simulink model "plant_model"  (R2024b)
settings: Solver=ode4  StartTime=0.0  StopTime=0.1  FixedStep=1e-6  RelTol=1e-3
libraries: spsSeriesRLCBranchLib x11, fuzblock x7, spsPWMGeneratorDCDCLib x7, spsFirstOrderFilterLib x4, spsIGBTDiodeLib x4, spsControlledVoltageSourceLib x3, spsCurrentMeasurementLib x3, spsGroundLib x3, spsVoltageMeasurementLib x3, spsIdealSwitchLib x2, SignalEditorBlockLib x2, spsDiodeLib x1
settings Model: Creator=Crisplan  LastModifiedBy=Crisplan
settings DataIOCC: ExternalInput=Input_Signals  LoadExternalInput=on

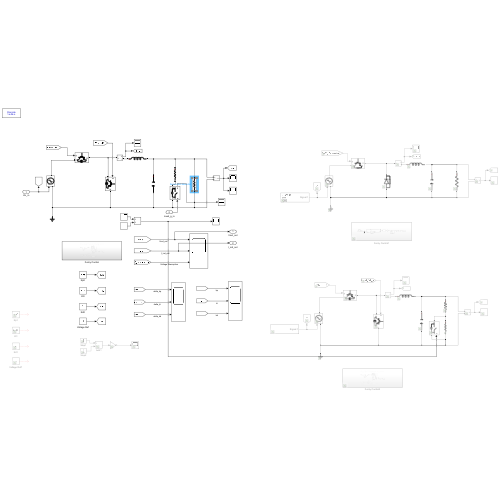
[thumbnail: Simulink's stored preview of the top-level diagram]
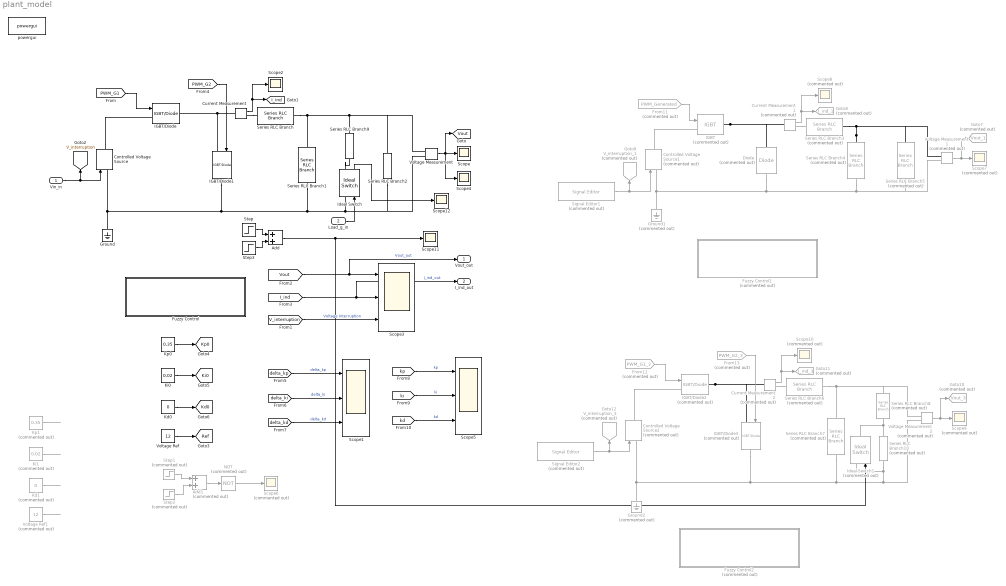
== system plant_model ==
  Vin_in : Inport
  Load_g_in : Inport  Port=2
  Add : Sum
  Add1 : Sum  Commented=on
  Controlled Voltage Source : spsControlledVoltageSourceLib/Controlled Voltage Source  Initialize=on  Source_Type=DC  Amplitude=0  Phase=0  Frequency=0  Measurements=None
  Controlled Voltage Source1 : spsControlledVoltageSourceLib/Controlled Voltage Source  Commented=on  Initialize=on  Source_Type=DC  Amplitude=0  Phase=0  Frequency=0  Measurements=None
  Controlled Voltage Source2 : spsControlledVoltageSourceLib/Controlled Voltage Source  Commented=on  Initialize=on  Source_Type=DC  Amplitude=0  Phase=0  Frequency=0  Measurements=None
  Current Measurement : spsCurrentMeasurementLib/Current Measurement  PhasorSimulation=off  OutputType=Complex  PSBequivalent=0
  Current Measurement1 : spsCurrentMeasurementLib/Current Measurement  Commented=on  PhasorSimulation=off  OutputType=Complex  PSBequivalent=0
  Current Measurement2 : spsCurrentMeasurementLib/Current Measurement  Commented=on  PhasorSimulation=off  OutputType=Complex  PSBequivalent=0
  Diode : spsDiodeLib/Diode  Commented=on  Ron=0.001  Lon=0  Vf=0.8  IC=0  UseSnubber=0  Rs=500  Cs=250e-9  Measurements=off
  From11 : From  Commented=on  GotoTag=PWM_Generated  TagVisibility=global
  From12 : From  Commented=on  GotoTag=PWM_G1_3  TagVisibility=global
  From13 : From  Commented=on  GotoTag=PWM_G2_3  TagVisibility=global
  Fuzzy Control : Subsystem
  Fuzzy Control1 : Subsystem  Commented=on
  Fuzzy Control2 : Subsystem  Commented=on
  Goto10 : Goto  Commented=on  GotoTag=Vout_3  TagVisibility=global
  Goto11 : Goto  Commented=on  GotoTag=I_ind_3  TagVisibility=global
  Goto12 : Goto  Commented=on  GotoTag=V_interruption_3  TagVisibility=global
  Goto7 : Goto  Commented=on  GotoTag=Vout_1  TagVisibility=global
  Goto8 : Goto  Commented=on  GotoTag=I_ind_1  TagVisibility=global
  Goto9 : Goto  Commented=on  GotoTag=V_interruption_1  TagVisibility=global
  Ground : spsGroundLib/Ground  LConnTagsString=a
  Ground1 : spsGroundLib/Ground  Commented=on  LConnTagsString=a
  Ground2 : spsGroundLib/Ground  Commented=on  LConnTagsString=a
  IGBT : spsIGBTLib/IGBT  Commented=on  Ron=0.001  Lon=0  Vf=1  Tf=1e-6  Tt=2e-6  IC=0  Rs=1e5  Cs=inf  Measurements=off
  IGBT/Diode : spsIGBTDiodeLib/IGBT//Diode  Ron=1e-3  Rs=1e5  Cs=inf  Measurements=off
  IGBT/Diode1 : spsIGBTDiodeLib/IGBT//Diode  Ron=1e-3  Rs=1e5  Cs=inf  Measurements=off
  IGBT/Diode2 : spsIGBTDiodeLib/IGBT//Diode  Commented=on  Ron=1e-3  Rs=1e5  Cs=inf  Measurements=off
  IGBT/Diode3 : spsIGBTDiodeLib/IGBT//Diode  Commented=on  Ron=1e-3  Rs=1e5  Cs=inf  Measurements=off
  Ideal Switch : spsIdealSwitchLib/Ideal Switch  Ron=1e-6  Lon=0  IC=0  Rs=1e5  Cs=inf  Measurements=on
  Ideal Switch1 : spsIdealSwitchLib/Ideal Switch  Commented=on  Ron=0.001  Lon=0  IC=0  Rs=1e5  Cs=inf  Measurements=off
  Kd0 : Constant  Value=0  SampleTime=1e-4
  Kd1 : Constant  Commented=on  Value=0  SampleTime=1e-4
  Ki0 : Constant  Value=0.02  SampleTime=1e-4
  Ki1 : Constant  Commented=on  Value=0.02  SampleTime=1e-4
  Kp0 : Constant  Value=0.35  SampleTime=1e-4
  Kp1 : Constant  Commented=on  Value=0.35  SampleTime=1e-4
  NOT : Logic  Commented=on  Operator=NOT  IconShape=distinctive  AllPortsSameDT=off  OutDataTypeStr=boolean
  Scope{,2,4,11..12} (5 alike) : Scope
  Scope1 : Scope  NumInputPorts=3
  Scope{6..10} (5 alike) : Scope  Commented=on
  Scope3 : Scope  NumInputPorts=3
  Scope5 : Scope  NumInputPorts=3
  Series RLC Branch : spsSeriesRLCBranchLib/Series RLC Branch  LConnTagsString=__new0  RConnTagsString=__new0  BranchType=L  Resistance=1  Inductance=0.015  SetiL0=off  InitialCurrent=0  Capacitance=1e-6  Setx0=off  InitialVoltage=0  Measurements=None
  Series RLC Branch1 : spsSeriesRLCBranchLib/Series RLC Branch  LConnTagsString=__new0  RConnTagsString=__new0  BranchType=C  Resistance=1  Inductance=1e-3  SetiL0=off  InitialCurrent=0  Capacitance=50e-6  Setx0=off  InitialVoltage=0  Measurements=None
  Series RLC Branch10 : spsSeriesRLCBranchLib/Series RLC Branch  Commented=on  LConnTagsString=__new0  RConnTagsString=__new0  BranchType=R  Resistance=2  Inductance=1e-3  SetiL0=off  InitialCurrent=0  Capacitance=1e-6  Setx0=off  InitialVoltage=0  Measurements=None
  Series RLC Branch2 : spsSeriesRLCBranchLib/Series RLC Branch  LConnTagsString=__new0  RConnTagsString=__new0  BranchType=R  Resistance=10  Inductance=1e-3  SetiL0=off  InitialCurrent=0  Capacitance=1e-6  Setx0=off  InitialVoltage=0  Measurements=None
  Series RLC Branch3 : spsSeriesRLCBranchLib/Series RLC Branch  Commented=on  LConnTagsString=__new0  RConnTagsString=__new0  BranchType=L  Resistance=1  Inductance=0.015  SetiL0=off  InitialCurrent=0  Capacitance=1e-6  Setx0=off  InitialVoltage=0  Measurements=None
  Series RLC Branch4 : spsSeriesRLCBranchLib/Series RLC Branch  Commented=on  LConnTagsString=__new0  RConnTagsString=__new0  BranchType=C  Resistance=1  Inductance=1e-3  SetiL0=off  InitialCurrent=0  Capacitance=50e-6  Setx0=off  InitialVoltage=0  Measurements=None
  Series RLC Branch5 : spsSeriesRLCBranchLib/Series RLC Branch  Commented=on  LConnTagsString=__new0  RConnTagsString=__new0  BranchType=R  Resistance=10  Inductance=1e-3  SetiL0=off  InitialCurrent=0  Capacitance=1e-6  Setx0=off  InitialVoltage=0  Measurements=None
  Series RLC Branch6 : spsSeriesRLCBranchLib/Series RLC Branch  Commented=on  LConnTagsString=__new0  RConnTagsString=__new0  BranchType=L  Resistance=1  Inductance=0.015  SetiL0=off  InitialCurrent=0  Capacitance=1e-6  Setx0=off  InitialVoltage=0  Measurements=None
  Series RLC Branch7 : spsSeriesRLCBranchLib/Series RLC Branch  Commented=on  LConnTagsString=__new0  RConnTagsString=__new0  BranchType=C  Resistance=1  Inductance=1e-3  SetiL0=off  InitialCurrent=0  Capacitance=50e-6  Setx0=off  InitialVoltage=0  Measurements=None
  Series RLC Branch8 : spsSeriesRLCBranchLib/Series RLC Branch  Commented=on  LConnTagsString=__new0  RConnTagsString=__new0  BranchType=R  Resistance=10  Inductance=1e-3  SetiL0=off  InitialCurrent=0  Capacitance=1e-6  Setx0=off  InitialVoltage=0  Measurements=None
  Series RLC Branch9 : spsSeriesRLCBranchLib/Series RLC Branch  LConnTagsString=__new0  RConnTagsString=__new0  BranchType=R  Resistance=10  Inductance=1e-3  SetiL0=off  InitialCurrent=0  Capacitance=1e-6  Setx0=off  InitialVoltage=0  Measurements=None
  Signal Editor1 : SignalEditorBlockLib/Signal Editor  Commented=on  FileName=Vin_signal.mat  ActiveScenario=Scenario  ActiveSignal=Voltage Interruption  IsBus=off  OutputBusObjectStr=Bus: BusObject  SampleTime=0  Interpolate=off  ZeroCross=off  OutputAfterFinalValue=Setting to zero  Unit=inherit  PreserveSignalName=on  ApplySigPropsToAllScenarios=on  ApplySigPropsToAllSignals=off
  Signal Editor2 : SignalEditorBlockLib/Signal Editor  Commented=on  FileName=data\Vin.mat  ActiveScenario=Scenario  ActiveSignal=Voltage Interruption  IsBus=off  OutputBusObjectStr=Bus: BusObject  SampleTime=0  Interpolate=off  ZeroCross=off  OutputAfterFinalValue=Setting to zero  Unit=inherit  PreserveSignalName=on  ApplySigPropsToAllScenarios=on  ApplySigPropsToAllSignals=off
  Step : Step  Time=0  SampleTime=0
  Step1 : Step  Commented=on  Time=0.02  SampleTime=0
  Step2 : Step  Commented=on  Time=0.07  After=-1  SampleTime=0
  Step3 : Step  Time=0.02  After=-1  SampleTime=0
  Voltage Measurement : spsVoltageMeasurementLib/Voltage Measurement  PhasorSimulation=off  OutputType=Complex  PSBequivalent=0
  Voltage Measurement1 : spsVoltageMeasurementLib/Voltage Measurement  Commented=on  PhasorSimulation=off  OutputType=Complex  PSBequivalent=0
  Voltage Measurement2 : spsVoltageMeasurementLib/Voltage Measurement  Commented=on  PhasorSimulation=off  OutputType=Complex  PSBequivalent=0
  Voltage Ref : Constant  Value=12  SampleTime=1e-4
  Voltage Ref1 : Constant  Commented=on  Value=12  SampleTime=1e-4
  powergui : spspowerguiLib/powergui  Priority=1  SimulationMode=Discrete  SampleTime=1e-6  frequency=60  Iterations=50  frequencyindice=0  Pbase=100e6  ErrMax=1e-4  UnitsV=kV  UnitsW=MW  buscounter=0  FunctionMessages=off  echomessages=off  EnableUseOfTLC=off  CurrentSourceSwitches=off  DisableSnubberDevices=off  DisableRonSwitches=off  DisableVfSwitches=off  DisplayEquations=off  AutomaticDiscreteSolvers=off  SolverType=Tustin/Backward Euler (TBE)  Interpol=off  ExternalGateDelay=off  methode=off  Ts=100  x0status=blocks  SPID=on  SwTol=0  HookPort=off  NonlinearTolerance=1e-4  nMaxIteration=100  ContinueOnMaxIteration=off  RestoreLinks=warning  ResistiveCurrentMeasurement=off  Frange=[0:2:500]  Ylog=off  Xlog=on  ShowGrid=off  save=off  variable=ZData  structure=0  ZoomFFT=off  StartTime=0.0  cycles=1  DisplayStyle=1  fundamental=60  FreqAxis=off  MaxFrequency=1000  frequencyindicesteady=1  RmsSteady=1  display=off
  Vout_out : Outport
  I_ind_out : Outport  Port=2
  tag scope: I_ind=global, Kd0=global, Ki0=global, Kp0=global, Ref=global, V_interruption=global, Vout=global
  wires:
  [I_ind] -> Scope3/2, I_ind_out/1  "I_ind_out"
  Voltage Measurement/1 -> Scope4/1, [Vout], Scope/1
  [V_interruption] -> Scope3/3  "Voltage Interruption"
  Vin_in/1 -> [V_interruption], Controlled Voltage Source/1
  [Vout] -> Scope3/1, Vout_out/1  "Vout_out"
  [PWM_G1] -> IGBT/Diode/1
  Current Measurement/1 -> Scope2/1, [I_ind]
  Voltage Ref/1 -> [Ref]
  Kp0/1 -> [Kp0]
  Ki0/1 -> [Ki0]
  Kd0/1 -> [Kd0]
  [PWM_G2] -> IGBT/Diode1/1
  [delta_ki] -> Scope1/2  "delta_ki"
  [delta_kp] -> Scope1/1  "delta_kp"
  [delta_kd] -> Scope1/3  "delta_kd"
  [kp] -> Scope5/1  "kp"
  [ki] -> Scope5/2  "ki"
  [kd] -> Scope5/3  "kd"
  Step1/1 -> Add1/1
  Step2/1 -> Add1/2
  Add1/1 -> NOT/1
  NOT/1 -> Scope6/1
  Signal Editor1/1 -> Goto9/1, Controlled Voltage Source1/1
  Voltage Measurement1/1 -> Goto7/1, Scope7/1
  From11/1 -> IGBT/1
  Current Measurement1/1 -> Scope8/1, Goto8/1
  Current Measurement2/1 -> Scope10/1, Goto11/1
  From13/1 -> IGBT/Diode3/1
  Voltage Measurement2/1 -> Goto10/1, Scope9/1
  From12/1 -> IGBT/Diode2/1
  Signal Editor2/1 -> Goto12/1, Controlled Voltage Source2/1
  Step/1 -> Add/1
  Step3/1 -> Add/2
  Kd1/1 -> ?
  Voltage Ref1/1 -> ?
  Kp1/1 -> ?
  Ki1/1 -> ?
  Add/1 -> Scope11/1, Ideal Switch1/1
  Ideal Switch/1 -> Scope12/1
  Load_g_in/1 -> Ideal Switch/1
  connections:
  Series RLC Branch9/LConn1 -- Series RLC Branch2/LConn1 -- Voltage Measurement/LConn1 -- Series RLC Branch1/LConn1 -- Series RLC Branch/RConn1
  Ground/LConn1 -- Series RLC Branch2/RConn1 -- Voltage Measurement/LConn2 -- Ideal Switch/LConn1 -- Series RLC Branch1/RConn1 -- IGBT/Diode1/RConn1 -- Controlled Voltage Source/LConn1
  Current Measurement/LConn1 -- IGBT/Diode1/LConn1 -- IGBT/Diode/RConn1
  IGBT/Diode/LConn1 -- Controlled Voltage Source/RConn1
  Current Measurement/RConn1 -- Series RLC Branch/LConn1
  Ground1/LConn1 -- Diode/LConn1 -- Voltage Measurement1/LConn2 -- Series RLC Branch5/RConn1 -- Series RLC Branch4/RConn1 -- Controlled Voltage Source1/LConn1
  Series RLC Branch4/LConn1 -- Series RLC Branch3/RConn1 -- Voltage Measurement1/LConn1 -- Series RLC Branch5/LConn1
  IGBT/RConn1 -- Diode/RConn1 -- Current Measurement1/LConn1
  IGBT/LConn1 -- Controlled Voltage Source1/RConn1
  Current Measurement1/RConn1 -- Series RLC Branch3/LConn1
  Series RLC Branch6/RConn1 -- Series RLC Branch7/LConn1 -- Voltage Measurement2/LConn1 -- Series RLC Branch8/LConn1
  Series RLC Branch10/RConn1 -- Ground2/LConn1 -- Controlled Voltage Source2/LConn1 -- IGBT/Diode3/RConn1 -- Series RLC Branch7/RConn1 -- Voltage Measurement2/LConn2 -- Ideal Switch1/LConn1
  IGBT/Diode2/RConn1 -- Current Measurement2/LConn1 -- IGBT/Diode3/LConn1
  IGBT/Diode2/LConn1 -- Controlled Voltage Source2/RConn1
  Current Measurement2/RConn1 -- Series RLC Branch6/LConn1
  Series RLC Branch10/LConn1 -- Series RLC Branch8/RConn1 -- Ideal Switch1/RConn1
  Ideal Switch/RConn1 -- Series RLC Branch9/RConn1

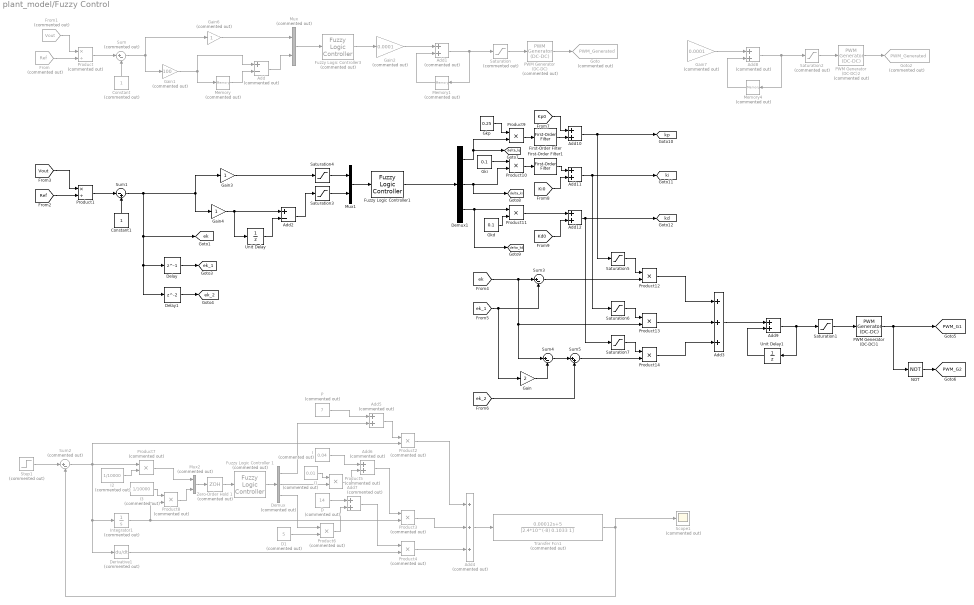
== system plant_model/Fuzzy Control ==
  Add : Sum  Commented=on  Inputs=+-
  Add{1,5..8} (5 alike) : Sum  Commented=on
  Add{9..12} (4 alike) : Sum
  Add2 : Sum  Inputs=+-
  Add3 : Sum  Inputs=+++
  Add4 : Sum  Commented=on  Inputs=+++
  Constant : Constant  Commented=on
  Constant1 : Constant  SampleTime=1e-4
  D : Constant  Commented=on  Value=14
  D1 : Constant  Commented=on  Value=5
  Delay : Delay  DelayLength=1  SampleTime=1e-4
  Delay1 : Delay  SampleTime=1e-4
  Demux : Demux  Commented=on  Outputs=3
  Demux1 : Demux  Outputs=3
  Derivative1 : Derivative  Commented=on
  First-Order Filter : spsFirstOrderFilterLib/First-Order Filter  FilterType=Lowpass  Tc=0.003  Ts=0  Initialize=on  Vac_Init=[0, 0, 60]  Vdc_Init=0  PlotResponse=off  FreqRange="[0,  200,  1]"
  First-Order Filter1 : spsFirstOrderFilterLib/First-Order Filter  FilterType=Lowpass  Tc=0.003  Ts=0  Initialize=on  Vac_Init=[0, 0, 60]  Vdc_Init=0  PlotResponse=off  FreqRange="[0,  200,  1]"
  From : From  Commented=on  GotoTag=Ref  TagVisibility=global
  From1 : From  Commented=on  GotoTag=Vout  TagVisibility=global
  Fuzzy Logic Controller 1 : fuzblock/Fuzzy Logic  Controller  Commented=on  FIS='FuzzyPID_Triangle_V1.fis'  OutputSampleNumber=101  DataType=double  FuzzifiedInputs=off  RuleFiringStrengths=off  RuleOutputs=off  AggregatedOutputs=off  SimulateUsing=Interpreted execution  OutOfRangeInputValueMessage=warning  NoRuleFiredMessage=warning  EmptyOutputFuzzySetMessage=warning
  Fuzzy Logic Controller1 : fuzblock/Fuzzy Logic  Controller  FIS=fuzzy_rules  OutputSampleNumber=101  DataType=double  FuzzifiedInputs=off  RuleFiringStrengths=off  RuleOutputs=off  AggregatedOutputs=off  SimulateUsing=Interpreted execution  OutOfRangeInputValueMessage=warning  NoRuleFiredMessage=warning  EmptyOutputFuzzySetMessage=warning
  Fuzzy Logic Controller3 : fuzblock/Fuzzy Logic  Controller  Commented=on  FIS=Fuzzy_1  OutputSampleNumber=101  DataType=double  FuzzifiedInputs=off  RuleFiringStrengths=off  RuleOutputs=off  AggregatedOutputs=off  SimulateUsing=Interpreted execution  OutOfRangeInputValueMessage=warning  NoRuleFiredMessage=warning  EmptyOutputFuzzySetMessage=warning
  Gain : Gain  Gain=2
  Gain1 : Gain  Commented=on  Gain=100
  Gain2 : Gain  Commented=on  Gain=0.0001
  Gain3 : Gain
  Gain4 : Gain
  Gain6 : Gain  Commented=on
  Gain7 : Gain  Commented=on  Gain=0.0001
  Gkd : Constant  Value=0.1  SampleTime=1e-4
  Gki : Constant  Value=0.1  SampleTime=1e-4
  Gkp : Constant  Value=0.25  SampleTime=1e-4
  Goto : Goto  Commented=on  GotoTag=PWM_Generated  TagVisibility=global
  Goto2 : Goto  Commented=on  GotoTag=PWM_Generated  TagVisibility=global
  I : Constant  Commented=on  Value=0.04
  I1 : Constant  Commented=on  Value=0.01
  I2 : Constant  Commented=on  Value=1/10000
  I3 : Constant  Commented=on  Value=1/10000
  Integrator1 : Integrator  Commented=on
  Memory : Memory  Commented=on  InheritSampleTime=on
  Memory1 : Memory  Commented=on  InheritSampleTime=on
  Memory4 : Memory  Commented=on  InheritSampleTime=on
  Mux : Mux  Commented=on  Inputs=2
  Mux1 : Mux  Inputs=2
  Mux2 : Mux  Commented=on  Inputs=2
  NOT : Logic  Operator=NOT  IconShape=distinctive  AllPortsSameDT=off  OutDataTypeStr=boolean
  P : Constant  Commented=on  Value=7
  PWM Generator (DC-DC) : spsPWMGeneratorDCDCLib/PWM Generator (DC-DC)  Commented=on  Fsw=5000  Ts=0
  PWM Generator (DC-DC)1 : spsPWMGeneratorDCDCLib/PWM Generator (DC-DC)  Fsw=1e4  Ts=0
  PWM Generator (DC-DC)2 : spsPWMGeneratorDCDCLib/PWM Generator (DC-DC)  Commented=on  Fsw=5000  Ts=0
  Product : Product  Commented=on  Inputs=*/
  Product1 : Product  Inputs=*/
  Product{9..14} (6 alike) : Product
  Product{2..8} (7 alike) : Product  Commented=on
  Saturation : Saturate  Commented=on  UpperLimit=1  LowerLimit=0
  Saturation1 : Saturate  UpperLimit=0.8  LowerLimit=0
  Saturation2 : Saturate  Commented=on  UpperLimit=1  LowerLimit=0
  Saturation3 : Saturate  UpperLimit=3  LowerLimit=-3
  Saturation4 : Saturate  UpperLimit=3  LowerLimit=-3
  Saturation5 : Saturate  UpperLimit=5  LowerLimit=-1
  Saturation6 : Saturate  UpperLimit=5  LowerLimit=-1
  Saturation7 : Saturate  UpperLimit=5  LowerLimit=-1
  Scope1 : Scope  Commented=on
  Step1 : Step  Commented=on  SampleTime=0
  Sum : Sum  Commented=on  Inputs=|+-
  Sum1 : Sum  Inputs=|-+
  Sum2 : Sum  Commented=on  Inputs=|+-
  Sum3 : Sum  Inputs=|+-
  Sum4 : Sum  Inputs=|+-
  Sum5 : Sum  Inputs=|++
  Transfer Fcn1 : TransferFcn  Commented=on  Numerator=[0.00012 5]  Denominator=[2.4*10^(-8) 0.1033 1]
  Unit Delay : UnitDelay  SampleTime=1e-4  HasFrameUpgradeWarning=on
  Unit Delay1 : UnitDelay  SampleTime=1e-4  HasFrameUpgradeWarning=on
  Zero-Order Hold 1 : ZeroOrderHold  Commented=on  SampleTime=-1
  tag scope: PWM_G1=global, PWM_G2=global, delta_kd=global, delta_ki=global, delta_kp=global, ek=global, ek_1=global, ek_2=global, kd=global, ki=global, kp=global
  wires:
  From1/1 -> Product/1
  Product/1 -> Sum/1
  Add/1 -> Mux/2
  Saturation/1 -> PWM Generator (DC-DC)/1
  Add1/1 -> Saturation/1, Memory1/1
  Fuzzy Logic Controller3/1 -> Gain2/1
  Gain1/1 -> Memory/1, Add/1
  Sum/1 -> Gain6/1, Gain1/1
  Gain2/1 -> Add1/1
  Memory1/1 -> Add1/2
  PWM Generator (DC-DC)/1 -> Goto/1
  Memory/1 -> Add/2
  Constant/1 -> Sum/2
  From/1 -> Product/2
  Mux/1 -> Fuzzy Logic Controller3/1
  Gain6/1 -> Mux/1
  Product1/1 -> Sum1/1
  Constant1/1 -> Sum1/2
  [Vout] -> Product1/1
  [Ref] -> Product1/2
  I2/1 -> Product7/2
  Zero-Order Hold 1/1 -> Fuzzy Logic Controller 1/1
  Add7/1 -> Product4/1
  Product7/1 -> Mux2/1
  Product4/1 -> Add4/3
  Product6/1 -> Add7/2
  Product3/1 -> Add4/2
  Transfer Fcn1/1 -> Scope1/1, Sum2/2
  Add6/1 -> Product3/1
  Fuzzy Logic Controller 1/1 -> Demux/1
  Step1/1 -> Sum2/1
  I3/1 -> Product8/1
  I1/1 -> Product5/1
  Demux/1 -> Add5/2
  I/1 -> Add6/1
  Product8/1 -> Mux2/2
  Add4/1 -> Transfer Fcn1/1
  Integrator1/1 -> Product8/2, Product3/2
  Demux/3 -> Product6/1
  Sum2/1 -> Derivative1/1, Integrator1/1, Product7/1, Product2/2
  Mux2/1 -> Zero-Order Hold 1/1
  Product2/1 -> Add4/1
  Demux/2 -> Product5/2
  P/1 -> Add5/1
  D/1 -> Add7/1
  Add5/1 -> Product2/1
  Product5/1 -> Add6/2
  D1/1 -> Product6/2
  Derivative1/1 -> Product4/2
  Saturation2/1 -> PWM Generator (DC-DC)2/1
  ? -> Gain7/1
  Memory4/1 -> Add8/2
  Add8/1 -> Saturation2/1, Memory4/1
  Gain7/1 -> Add8/1
  PWM Generator (DC-DC)2/1 -> Goto2/1
  Fuzzy Logic Controller1/1 -> Demux1/1
  Delay/1 -> [ek_1]
  Delay1/1 -> [ek_2]
  Gkp/1 -> Product9/1
  Demux1/1 -> [delta_kp], Product9/2
  Gki/1 -> Product10/1
  Demux1/2 -> [delta_ki], Product10/2
  Gkd/1 -> Product11/2
  Demux1/3 -> [delta_kd], Product11/1
  [ek] -> Sum4/1, Product13/2, Sum3/1
  [ek_1] -> Gain/1, Sum3/2
  Sum3/1 -> Product12/2
  Gain/1 -> Sum4/2
  Sum4/1 -> Sum5/1
  [ek_2] -> Sum5/2
  Sum5/1 -> Product14/2
  Product12/1 -> Add3/1
  Product13/1 -> Add3/2
  Product14/1 -> Add3/3
  Add3/1 -> Add9/1
  Add9/1 -> Unit Delay1/1, Saturation1/1
  [Kp0] -> Add10/1
  [Ki0] -> Add11/2
  Product11/1 -> Add12/1
  [Kd0] -> Add12/2
  Add10/1 -> [kp], Saturation5/1
  Add11/1 -> [ki], Saturation6/1
  Add12/1 -> [kd], Saturation7/1
  Saturation1/1 -> PWM Generator (DC-DC)1/1
  PWM Generator (DC-DC)1/1 -> NOT/1, [PWM_G1]
  NOT/1 -> [PWM_G2]
  Sum1/1 -> Gain4/1, Gain3/1, Delay1/1, Delay/1, [ek]
  Mux1/1 -> Fuzzy Logic Controller1/1
  Gain4/1 -> Unit Delay/1, Add2/1
  Add2/1 -> Saturation3/1
  Unit Delay1/1 -> Add9/2
  Product9/1 -> First-Order Filter/1
  First-Order Filter/1 -> Add10/2
  Product10/1 -> First-Order Filter1/1
  First-Order Filter1/1 -> Add11/1
  Saturation3/1 -> Mux1/2
  Gain3/1 -> Saturation4/1
  Saturation4/1 -> Mux1/1
  Saturation5/1 -> Product12/1
  Saturation6/1 -> Product13/1
  Saturation7/1 -> Product14/1
  Unit Delay/1 -> Add2/2

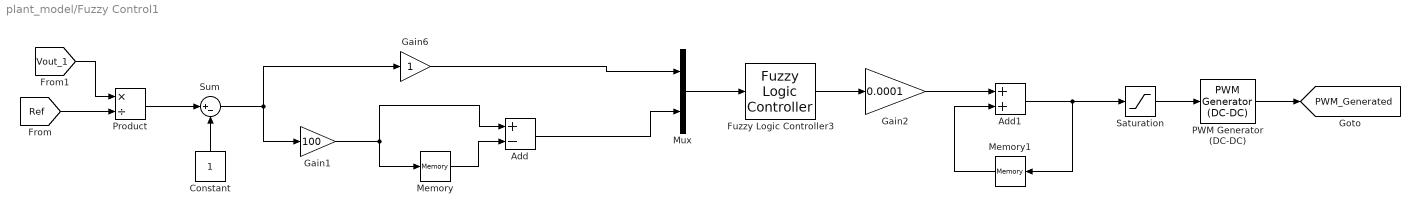
== system plant_model/Fuzzy Control1 ==
  Add : Sum  Inputs=+-
  Add1 : Sum
  Constant : Constant
  Fuzzy Logic Controller3 : fuzblock/Fuzzy Logic  Controller  FIS=Fuzzy_1  OutputSampleNumber=101  DataType=double  FuzzifiedInputs=off  RuleFiringStrengths=off  RuleOutputs=off  AggregatedOutputs=off  SimulateUsing=Interpreted execution  OutOfRangeInputValueMessage=warning  NoRuleFiredMessage=warning  EmptyOutputFuzzySetMessage=warning
  Gain1 : Gain  Gain=100
  Gain2 : Gain  Gain=0.0001
  Gain6 : Gain
  Memory : Memory  InheritSampleTime=on
  Memory1 : Memory  InheritSampleTime=on
  Mux : Mux  Inputs=2
  PWM Generator (DC-DC) : spsPWMGeneratorDCDCLib/PWM Generator (DC-DC)  Fsw=5000  Ts=0
  Product : Product  Inputs=*/
  Saturation : Saturate  UpperLimit=1  LowerLimit=0
  Sum : Sum  Inputs=|+-
  tag scope: PWM_Generated=global
  wires:
  [Vout_1] -> Product/1
  Product/1 -> Sum/1
  Saturation/1 -> PWM Generator (DC-DC)/1
  Add1/1 -> Saturation/1, Memory1/1
  Fuzzy Logic Controller3/1 -> Gain2/1
  Gain1/1 -> Memory/1, Add/1
  Sum/1 -> Gain6/1, Gain1/1
  Gain2/1 -> Add1/1
  Memory1/1 -> Add1/2
  PWM Generator (DC-DC)/1 -> [PWM_Generated]
  Memory/1 -> Add/2
  Constant/1 -> Sum/2
  [Ref] -> Product/2
  Mux/1 -> Fuzzy Logic Controller3/1
  Gain6/1 -> Mux/1
  Add/1 -> Mux/2

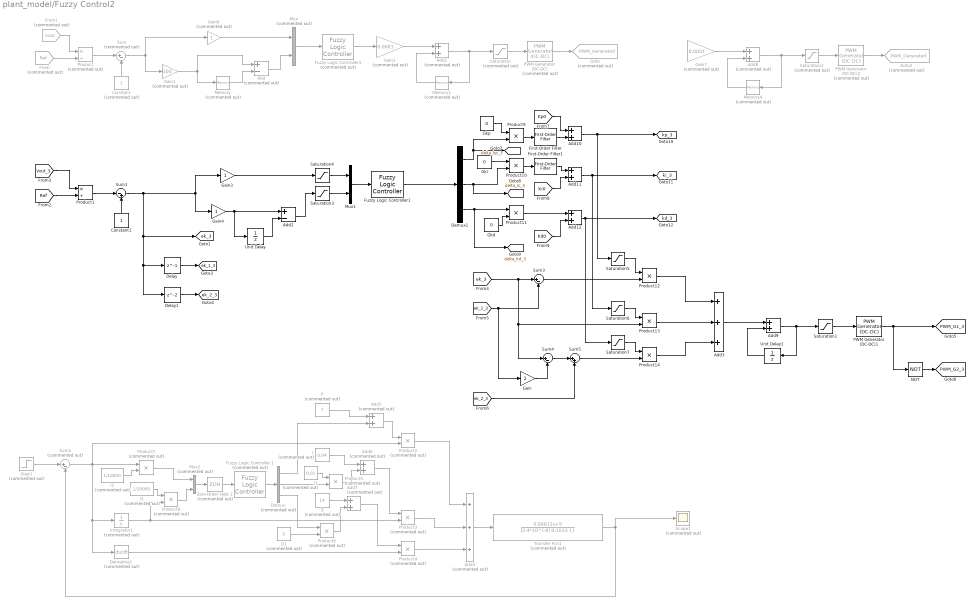
== system plant_model/Fuzzy Control2 ==
  Add : Sum  Commented=on  Inputs=+-
  Add{1,5..8} (5 alike) : Sum  Commented=on
  Add{9..12} (4 alike) : Sum
  Add2 : Sum  Inputs=+-
  Add3 : Sum  Inputs=+++
  Add4 : Sum  Commented=on  Inputs=+++
  Constant : Constant  Commented=on
  Constant1 : Constant  SampleTime=1e-4
  D : Constant  Commented=on  Value=14
  D1 : Constant  Commented=on  Value=5
  Delay : Delay  DelayLength=1  SampleTime=1e-4
  Delay1 : Delay  SampleTime=1e-4
  Demux : Demux  Commented=on  Outputs=3
  Demux1 : Demux  Outputs=3
  Derivative1 : Derivative  Commented=on
  First-Order Filter : spsFirstOrderFilterLib/First-Order Filter  FilterType=Lowpass  Tc=0.003  Ts=0  Initialize=on  Vac_Init=[0, 0, 60]  Vdc_Init=0  PlotResponse=off  FreqRange="[0,  200,  1]"
  First-Order Filter1 : spsFirstOrderFilterLib/First-Order Filter  FilterType=Lowpass  Tc=0.003  Ts=0  Initialize=on  Vac_Init=[0, 0, 60]  Vdc_Init=0  PlotResponse=off  FreqRange="[0,  200,  1]"
  From : From  Commented=on  GotoTag=Ref  TagVisibility=global
  From1 : From  Commented=on  GotoTag=Vout  TagVisibility=global
  Fuzzy Logic Controller 1 : fuzblock/Fuzzy Logic  Controller  Commented=on  FIS='FuzzyPID_Triangle_V1.fis'  OutputSampleNumber=101  DataType=double  FuzzifiedInputs=off  RuleFiringStrengths=off  RuleOutputs=off  AggregatedOutputs=off  SimulateUsing=Interpreted execution  OutOfRangeInputValueMessage=warning  NoRuleFiredMessage=warning  EmptyOutputFuzzySetMessage=warning
  Fuzzy Logic Controller1 : fuzblock/Fuzzy Logic  Controller  FIS=fuzzy_rules  OutputSampleNumber=101  DataType=double  FuzzifiedInputs=off  RuleFiringStrengths=off  RuleOutputs=off  AggregatedOutputs=off  SimulateUsing=Interpreted execution  OutOfRangeInputValueMessage=warning  NoRuleFiredMessage=warning  EmptyOutputFuzzySetMessage=warning
  Fuzzy Logic Controller3 : fuzblock/Fuzzy Logic  Controller  Commented=on  FIS=Fuzzy_1  OutputSampleNumber=101  DataType=double  FuzzifiedInputs=off  RuleFiringStrengths=off  RuleOutputs=off  AggregatedOutputs=off  SimulateUsing=Interpreted execution  OutOfRangeInputValueMessage=warning  NoRuleFiredMessage=warning  EmptyOutputFuzzySetMessage=warning
  Gain : Gain  Gain=2
  Gain1 : Gain  Commented=on  Gain=100
  Gain2 : Gain  Commented=on  Gain=0.0001
  Gain3 : Gain
  Gain4 : Gain
  Gain6 : Gain  Commented=on
  Gain7 : Gain  Commented=on  Gain=0.0001
  Gkd : Constant  Value=0  SampleTime=1e-4
  Gki : Constant  Value=0  SampleTime=1e-4
  Gkp : Constant  Value=0  SampleTime=1e-4
  Goto : Goto  Commented=on  GotoTag=PWM_Generated  TagVisibility=global
  Goto2 : Goto  Commented=on  GotoTag=PWM_Generated  TagVisibility=global
  I : Constant  Commented=on  Value=0.04
  I1 : Constant  Commented=on  Value=0.01
  I2 : Constant  Commented=on  Value=1/10000
  I3 : Constant  Commented=on  Value=1/10000
  Integrator1 : Integrator  Commented=on
  Memory : Memory  Commented=on  InheritSampleTime=on
  Memory1 : Memory  Commented=on  InheritSampleTime=on
  Memory4 : Memory  Commented=on  InheritSampleTime=on
  Mux : Mux  Commented=on  Inputs=2
  Mux1 : Mux  Inputs=2
  Mux2 : Mux  Commented=on  Inputs=2
  NOT : Logic  Operator=NOT  IconShape=distinctive  AllPortsSameDT=off  OutDataTypeStr=boolean
  P : Constant  Commented=on  Value=7
  PWM Generator (DC-DC) : spsPWMGeneratorDCDCLib/PWM Generator (DC-DC)  Commented=on  Fsw=5000  Ts=0
  PWM Generator (DC-DC)1 : spsPWMGeneratorDCDCLib/PWM Generator (DC-DC)  Fsw=1e4  Ts=0
  PWM Generator (DC-DC)2 : spsPWMGeneratorDCDCLib/PWM Generator (DC-DC)  Commented=on  Fsw=5000  Ts=0
  Product : Product  Commented=on  Inputs=*/
  Product1 : Product  Inputs=*/
  Product{9..14} (6 alike) : Product
  Product{2..8} (7 alike) : Product  Commented=on
  Saturation : Saturate  Commented=on  UpperLimit=1  LowerLimit=0
  Saturation1 : Saturate  UpperLimit=0.8  LowerLimit=0
  Saturation2 : Saturate  Commented=on  UpperLimit=1  LowerLimit=0
  Saturation3 : Saturate  UpperLimit=3  LowerLimit=-3
  Saturation4 : Saturate  UpperLimit=3  LowerLimit=-3
  Saturation5 : Saturate  UpperLimit=5  LowerLimit=-1
  Saturation6 : Saturate  UpperLimit=5  LowerLimit=-1
  Saturation7 : Saturate  UpperLimit=5  LowerLimit=-1
  Scope1 : Scope  Commented=on
  Step1 : Step  Commented=on  SampleTime=0
  Sum : Sum  Commented=on  Inputs=|+-
  Sum1 : Sum  Inputs=|-+
  Sum2 : Sum  Commented=on  Inputs=|+-
  Sum3 : Sum  Inputs=|+-
  Sum4 : Sum  Inputs=|+-
  Sum5 : Sum  Inputs=|++
  Transfer Fcn1 : TransferFcn  Commented=on  Numerator=[0.00012 5]  Denominator=[2.4*10^(-8) 0.1033 1]
  Unit Delay : UnitDelay  SampleTime=1e-4  HasFrameUpgradeWarning=on
  Unit Delay1 : UnitDelay  SampleTime=1e-4  HasFrameUpgradeWarning=on
  Zero-Order Hold 1 : ZeroOrderHold  Commented=on  SampleTime=-1
  tag scope: PWM_G1_3=global, PWM_G2_3=global, delta_kd_3=global, delta_ki_3=global, delta_kp_3=global, ek_1_3=global, ek_2_3=global, ek_3=global, kd_3=global, ki_3=global, kp_3=global
  wires:
  From1/1 -> Product/1
  Product/1 -> Sum/1
  Add/1 -> Mux/2
  Saturation/1 -> PWM Generator (DC-DC)/1
  Add1/1 -> Saturation/1, Memory1/1
  Fuzzy Logic Controller3/1 -> Gain2/1
  Gain1/1 -> Memory/1, Add/1
  Sum/1 -> Gain6/1, Gain1/1
  Gain2/1 -> Add1/1
  Memory1/1 -> Add1/2
  PWM Generator (DC-DC)/1 -> Goto/1
  Memory/1 -> Add/2
  Constant/1 -> Sum/2
  From/1 -> Product/2
  Mux/1 -> Fuzzy Logic Controller3/1
  Gain6/1 -> Mux/1
  Product1/1 -> Sum1/1
  Constant1/1 -> Sum1/2
  [Vout_3] -> Product1/1
  [Ref] -> Product1/2
  I2/1 -> Product7/2
  Zero-Order Hold 1/1 -> Fuzzy Logic Controller 1/1
  Add7/1 -> Product4/1
  Product7/1 -> Mux2/1
  Product4/1 -> Add4/3
  Product6/1 -> Add7/2
  Product3/1 -> Add4/2
  Transfer Fcn1/1 -> Scope1/1, Sum2/2
  Add6/1 -> Product3/1
  Fuzzy Logic Controller 1/1 -> Demux/1
  Step1/1 -> Sum2/1
  I3/1 -> Product8/1
  I1/1 -> Product5/1
  Demux/1 -> Add5/2
  I/1 -> Add6/1
  Product8/1 -> Mux2/2
  Add4/1 -> Transfer Fcn1/1
  Integrator1/1 -> Product8/2, Product3/2
  Demux/3 -> Product6/1
  Sum2/1 -> Derivative1/1, Integrator1/1, Product7/1, Product2/2
  Mux2/1 -> Zero-Order Hold 1/1
  Product2/1 -> Add4/1
  Demux/2 -> Product5/2
  P/1 -> Add5/1
  D/1 -> Add7/1
  Add5/1 -> Product2/1
  Product5/1 -> Add6/2
  D1/1 -> Product6/2
  Derivative1/1 -> Product4/2
  Saturation2/1 -> PWM Generator (DC-DC)2/1
  ? -> Gain7/1
  Memory4/1 -> Add8/2
  Add8/1 -> Saturation2/1, Memory4/1
  Gain7/1 -> Add8/1
  PWM Generator (DC-DC)2/1 -> Goto2/1
  Fuzzy Logic Controller1/1 -> Demux1/1
  Delay/1 -> [ek_1_3]
  Delay1/1 -> [ek_2_3]
  Gkp/1 -> Product9/1
  Demux1/1 -> [delta_kp_3], Product9/2
  Gki/1 -> Product10/1
  Demux1/2 -> [delta_ki_3], Product10/2
  Gkd/1 -> Product11/2
  Demux1/3 -> [delta_kd_3], Product11/1
  [ek_3] -> Sum4/1, Product13/2, Sum3/1
  [ek_1_3] -> Gain/1, Sum3/2
  Sum3/1 -> Product12/2
  Gain/1 -> Sum4/2
  Sum4/1 -> Sum5/1
  [ek_2_3] -> Sum5/2
  Sum5/1 -> Product14/2
  Product12/1 -> Add3/1
  Product13/1 -> Add3/2
  Product14/1 -> Add3/3
  Add3/1 -> Add9/1
  Add9/1 -> Unit Delay1/1, Saturation1/1
  [Kp0] -> Add10/1
  [Ki0] -> Add11/2
  Product11/1 -> Add12/1
  [Kd0] -> Add12/2
  Add10/1 -> [kp_3], Saturation5/1
  Add11/1 -> [ki_3], Saturation6/1
  Add12/1 -> [kd_3], Saturation7/1
  Saturation1/1 -> PWM Generator (DC-DC)1/1
  PWM Generator (DC-DC)1/1 -> NOT/1, [PWM_G1_3]
  NOT/1 -> [PWM_G2_3]
  Sum1/1 -> Gain4/1, Gain3/1, Delay1/1, Delay/1, [ek_3]
  Mux1/1 -> Fuzzy Logic Controller1/1
  Gain4/1 -> Unit Delay/1, Add2/1
  Add2/1 -> Saturation3/1
  Unit Delay1/1 -> Add9/2
  Product9/1 -> First-Order Filter/1
  First-Order Filter/1 -> Add10/2
  Product10/1 -> First-Order Filter1/1
  First-Order Filter1/1 -> Add11/1
  Saturation3/1 -> Mux1/2
  Gain3/1 -> Saturation4/1
  Saturation4/1 -> Mux1/1
  Saturation5/1 -> Product12/1
  Saturation6/1 -> Product13/1
  Saturation7/1 -> Product14/1
  Unit Delay/1 -> Add2/2
